simulink model "pt3_simulation"  (R2020b)
settings: Solver=FixedStepAuto  StartTime=0.0  StopTime=1  FixedStep=T  RelTol=1e-3
settings Model: Creator=EAL  LastModifiedBy=EAL

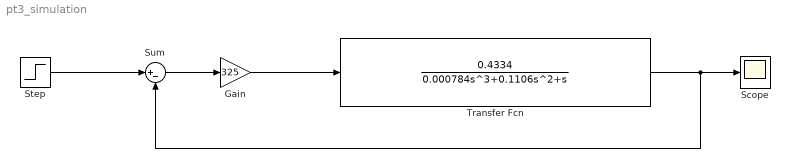
== system pt3_simulation ==
  Gain : Gain  Gain=325
  Scope : Scope
  Step : Step  Time=0  SampleTime=0
  Sum : Sum  Inputs=|+-
  Transfer Fcn : TransferFcn  Numerator=[0.4334]  Denominator="[0.000784  0.1106  1 0]"
  wires:
  Sum/1 -> Gain/1
  Step/1 -> Sum/1
  Gain/1 -> Transfer Fcn/1
  Transfer Fcn/1 -> Sum/2, Scope/1
